simulink model "Bidirectional_AC_DC_full_control_V0_5_book"  (R2024a)
settings: Solver=VariableStepAuto  StartTime=0.0  StopTime=10.0  FixedStep=1e-6  MaxStep=1e-6  RelTol=1e-3
libraries: spsSeriesRLCBranchLib x7, simulink x7, spsBreakerLib x6, spsVoltageMeasurementLib x4, spsMosfetLib x4, spsCurrentMeasurementLib x3, slpidlib x3, spsFirstOrderFilterLib x2, spsACVoltageSourceLib x1, spsAlphaBetaZerotodq0Lib x1, spsDCVoltageSourceLib x1, sps_lib x1
settings Model: Creator=MANSY  LastModifiedBy=MANSY

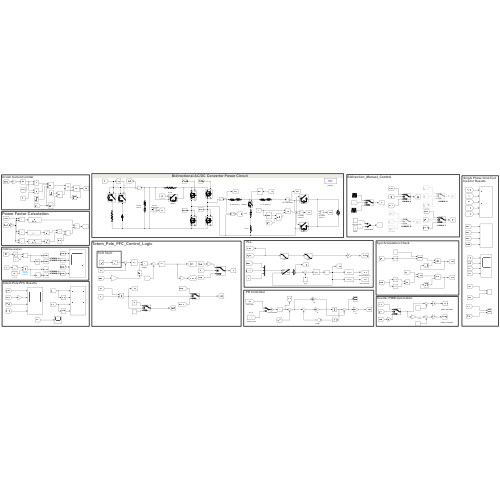
[thumbnail: Simulink's stored preview of the top-level diagram]
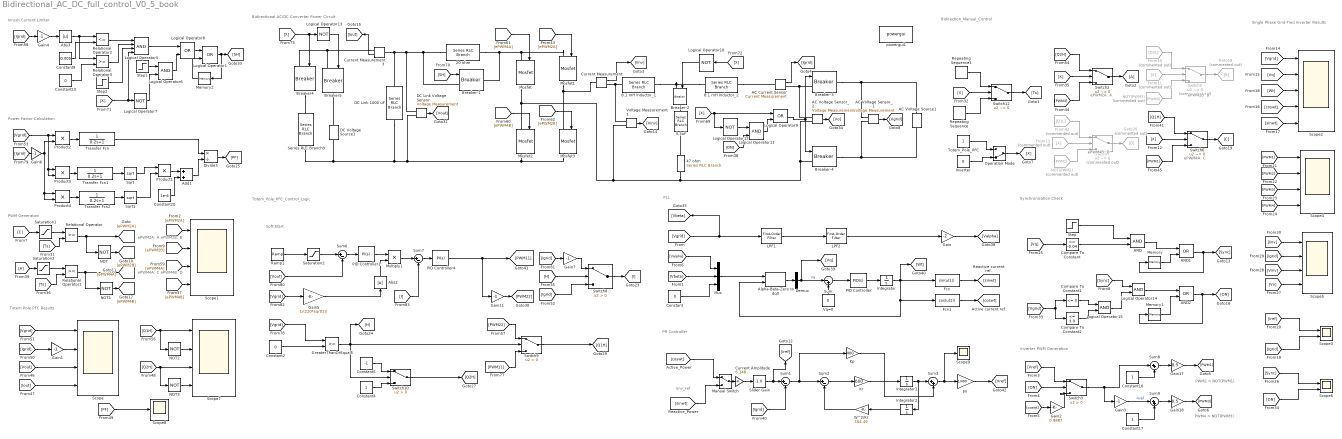
== system Bidirectional_AC_DC_full_control_V0_5_book ==
  note: Bidirectional AC/DC Converter Power Circuit
  note: Inrush Current Limiter
  note: Soft Start
  note: Power Factor Calculation
  note: Totem_Pole_PFC_Control_Logic
  note: PR Controller
  note: Synchronization Check
  note: Iinv_ref
  note: PLL
  note: Single Phase Grid-Tied
      |  Inverter Results
  note: Bidirection_Manual_Control
  note: ePWM2B: B
  note: ePWM2A: A
  note: ePWM4A: C
  note: ePWM4B: D
  note: PWM Generation
  note: PWM4 = NOT(PWM3)
  note: ePWM2A: A
      | ePWM2B: B
  note: ePWM4A: C
      | ePWM4B: D
  note: PWM2 = NOT(PWM1)
  note: Inverter PWM Generation
  note: Totem Pole PFC Results
  "          Totem_Pole_PFC" : Constant  OutDataTypeStr=boolean  SampleTime=1e-6
  20 ohm : spsSeriesRLCBranchLib/Series RLC Branch  LConnTagsString=__new0  RConnTagsString=__new0  BranchType=R  Resistance=20  Inductance=8.1e-3  SetiL0=off  InitialCurrent=0  Capacitance=1e-6  Setx0=off  InitialVoltage=0  Measurements=None
  3.3uF : spsSeriesRLCBranchLib/Series RLC Branch  LConnTagsString=__new0  RConnTagsString=__new0  BranchType=C  Resistance=30  Inductance=1e-3  SetiL0=off  InitialCurrent=0  Capacitance=3.3e-6  Setx0=off  InitialVoltage=0  Measurements=None
  47 ohm : spsSeriesRLCBranchLib/Series RLC Branch  LConnTagsString=__new0  RConnTagsString=__new0  BranchType=R  Resistance=40  Inductance=1e-3  SetiL0=off  InitialCurrent=0  Capacitance=3.3e-6  Setx0=off  InitialVoltage=0  Measurements=None
  8.1 mH Inductor_1 : spsSeriesRLCBranchLib/Series RLC Branch  LConnTagsString=__new0  RConnTagsString=__new0  BranchType=RL  Resistance=.001  Inductance=8e-3  SetiL0=off  InitialCurrent=0  Capacitance=1e-6  Setx0=off  InitialVoltage=0  Measurements=None
  8.1 mH Inductor_2 : spsSeriesRLCBranchLib/Series RLC Branch  LConnTagsString=__new0  RConnTagsString=__new0  BranchType=RL  Resistance=.001  Inductance=8e-3  SetiL0=off  InitialCurrent=0  Capacitance=1e-6  Setx0=off  InitialVoltage=0  Measurements=None
  AC Current Sensor : spsCurrentMeasurementLib/Current Measurement  PhasorSimulation=off  OutputType=Complex  PSBequivalent=0
  AC Voltage Sensor_1 : spsVoltageMeasurementLib/Voltage Measurement  PhasorSimulation=off  OutputType=Complex  PSBequivalent=0
  AC Voltage Sensor_2 : spsVoltageMeasurementLib/Voltage Measurement  PhasorSimulation=off  OutputType=Complex  PSBequivalent=0
  AC Voltage Source1 : spsACVoltageSourceLib/AC Voltage Source  Amplitude=230*sqrt(2)  Phase=0  Frequency=50  SampleTime=0  Measurements=None  BusType=swing  Pref=10e3  Qref=0  Qmin=-inf  Qmax=+inf
  AND : Logic  AllPortsSameDT=off  OutDataTypeStr=boolean
  AND1 : Logic  Operator=OR  AllPortsSameDT=off  OutDataTypeStr=boolean
  AND2 : Logic  Operator=OR  AllPortsSameDT=off  OutDataTypeStr=boolean
  Abs2 : Abs  SaturateOnIntegerOverflow=off
  Abs3 : Abs  SaturateOnIntegerOverflow=off
  Add1 : Sum
  Alpha-Beta-Zero to dq0 : spsAlphaBetaZerotodq0Lib/Alpha-Beta-Zero to dq0  Alignment=90 degrees behind phase A axis
  Breaker-{1..4} (4 alike) : spsBreakerLib/Breaker  InitialState=0  SwitchingTimes="[1/60  5/60]"  External=on  BreakerResistance=0.01  SnubberResistance=1e6  SnubberCapacitance=inf  Measurements=None  MoreParameters=on  NoBreakLoop=off
  Breaker4 : spsBreakerLib/Breaker  InitialState=0  SwitchingTimes="[1/60  5/60]"  External=on  BreakerResistance=0.01  SnubberResistance=1e6  SnubberCapacitance=inf  Measurements=None  MoreParameters=on  NoBreakLoop=off
  Breaker5 : spsBreakerLib/Breaker  InitialState=0  SwitchingTimes="[1/60  5/60]"  External=on  BreakerResistance=0.01  SnubberResistance=1e6  SnubberCapacitance=inf  Measurements=None  MoreParameters=on  NoBreakLoop=off
  Compare To Constant : simulink/Logic and Bit Operations/Compare To Constant  relop=>=  const=-0.04  OutDataTypeStr=boolean
  Compare To Constant1 : simulink/Logic and Bit Operations/Compare To Constant  relop=<=  const=0  OutDataTypeStr=boolean
  Compare To Constant2 : simulink/Logic and Bit Operations/Compare To Constant  relop=<=  const=3.0  OutDataTypeStr=boolean
  Constant : Constant  Value=0
  Constant10 : Constant  Value=0
  Constant16 : Constant
  Constant17 : Constant
  Constant2 : Constant  Value=0
  Constant20 : Constant  Value=1e-6
  Constant4 : Constant
  Constant5 : Constant  Value=-1
  Constant9 : Constant  Value=0.005
  Current Amplitude : Gain  Gain=6.148
  Current Measurement : spsCurrentMeasurementLib/Current Measurement  PhasorSimulation=off  OutputType=Complex  PSBequivalent=0
  Current Measurement3 : spsCurrentMeasurementLib/Current Measurement  PhasorSimulation=off  OutputType=Complex  PSBequivalent=0
  DC Link 1000 uF : spsSeriesRLCBranchLib/Series RLC Branch  LConnTagsString=__new0  RConnTagsString=__new0  BranchType=RC  Resistance=.0042  Inductance=1e-3  SetiL0=off  InitialCurrent=0  Capacitance=1000e-6  Setx0=off  InitialVoltage=400  Measurements=None
  DC Link Voltage Sensor : spsVoltageMeasurementLib/Voltage Measurement  PhasorSimulation=off  OutputType=Complex  PSBequivalent=0
  DC Voltage Source1 : spsDCVoltageSourceLib/DC Voltage Source  Amplitude=400  Measurements=None
  Demux : Demux  Outputs=3
  Divide3 : Product  Inputs=*/
  Fcn : Fcn  Expr=sin(u(1))
  Fcn1 : Fcn  Expr=cos(u(1))
  From10 : From  Commented=on  GotoTag=Q2L
  From11 : From  Commented=on  GotoTag=X
  From13 : From  Commented=on  GotoTag=X
  From39 : From
  From42 : From  Commented=on  GotoTag=Q1L
  Gain : Gain  Gain=-2
  Gain{1,3..4,6..7,11} (6 alike) : Gain  Gain=-1
  Gain17 : Gain  Gain=0.5
  Gain18 : Gain  Gain=0.5
  Gain2 : Gain  Gain=0.8887
  Gain5 : Gain  Gain=1/(220*sqrt(2))
  Goto18 : Goto  Commented=on  GotoTag=B
  Goto2 : Goto
  Goto20 : Goto  Commented=on  GotoTag=D
  GreaterThanOrEqual5 : RelationalOperator  OutDataTypeStr=boolean  RndMeth=Simplest  InputSameDT=off
  Integrator : Integrator
  Integrator1 : Integrator
  Integrator2 : Integrator
  Inverter : Constant  Value=0  OutDataTypeStr=boolean  SampleTime=1e-6
  Kp : Gain  Gain=400
  Kr : Gain  Gain=600
  LPF1 : spsFirstOrderFilterLib/First-Order Filter  FilterType=Lowpass  Tc=1/(2*pi*50)  Ts=0  Initialize=off  Vac_Init=[0, 0, 60]  Vdc_Init=0  PlotResponse=off  FreqRange="[0,  200,  1]"
  LPF2 : spsFirstOrderFilterLib/First-Order Filter  FilterType=Lowpass  Tc=1/(2*pi*50)  Ts=0  Initialize=off  Vac_Init=[0, 0, 60]  Vdc_Init=0  PlotResponse=off  FreqRange="[0,  200,  1]"
  Logical Operator1 : Logic  Operator=OR  AllPortsSameDT=off  OutDataTypeStr=boolean
  Logical Operator{7,10,12..13} (4 alike) : Logic  Operator=NOT  AllPortsSameDT=off  OutDataTypeStr=boolean
  Logical Operator{6,11,14..15} (4 alike) : Logic  AllPortsSameDT=off  OutDataTypeStr=boolean
  Logical Operator5 : Logic  Inputs=4  AllPortsSameDT=off  OutDataTypeStr=boolean
  Logical Operator8 : Logic  Operator=OR  AllPortsSameDT=off  OutDataTypeStr=boolean
  Logical Operator9 : Logic  Operator=OR  AllPortsSameDT=off  OutDataTypeStr=boolean
  Manual Switch : ManualSwitch
  Memory : Memory
  Memory1 : Memory
  Memory2 : Memory
  Mosfet{,1..3} (4 alike) : spsMosfetLib/Mosfet  Ron=0.1  Lon=0  Rd=0.01  Vfd=0  IC=0  Rs=1e5  Cs=inf  Measurements=on
  Multiply1 : Product
  Mux : Mux  Inputs=3
  NOT{,1..3} (4 alike) : Logic  Operator=NOT  AllPortsSameDT=off  OutDataTypeStr=boolean
  NOT(PWM1) : From  Commented=on  GotoTag=PWM2
  NOT(PWM3) : From  Commented=on  GotoTag=PWM4
  Operation Mode : ManualSwitch  CurrentSetting=0
  PID Controller : slpidlib/PID Controller  Controller=PID  Form=Parallel  TimeDomain=Continuous-time  UseExternalTs=off  SampleTime=-1  IntegratorMethod=Forward Euler  FilterMethod=Forward Euler  ControllerParametersSource=internal  P=100  I=10000  UseKiTs=off  D=0  UseExternalDerivativeSource=off  N=100  UseFilter=on  TunerSelectOption=Transfer Function Based (PID Tuner App)  InitialConditionSource=internal  InitialConditionForIntegrator=0  InitialConditionForFilter=0  DifferentiatorICPrevScaledInput=0  ExternalReset=none  TrackingMode=off  Kt=1  LimitOutput=off  SatLimitsSource=internal  UpperSaturationLimit=inf  LowerSaturationLimit=-inf  LinearizeAsGain=on  AntiWindupMode=none  Kb=1  LimitIntegrator=off  UpperIntegratorSaturationLimit=inf  LowerIntegratorSaturationLimit=-inf  POutMin=[]  POutMax=[]  IOutMin=[]  IOutMax=[]  DOutMin=[]  DOutMax=[]  NOutMin=[]  NOutMax=[]  SumOutMin=[]  SumOutMax=[]  SaturationOutMin=[]  SaturationOutMax=[]  PParamMin=[]  PParamMax=[]  IParamMin=[]  IParamMax=[]  DParamMin=[]  DParamMax=[]  NParamMin=[]  NParamMax=[]  KbParamMin=[]  KbParamMax=[]  KtParamMin=[]  KtParamMax=[]  KbOutMin=[]  KbOutMax=[]  KtOutMin=[]  KtOutMax=[]  IntegratorOutMin=[]  IntegratorOutMax=[]  FilterOutMin=[]  FilterOutMax=[]  SumI1OutMin=[]  SumI1OutMax=[]  SumI2OutMin=[]  SumI2OutMax=[]  SumI3OutMin=[]  SumI3OutMax=[]  SumI4OutMin=[]  SumI4OutMax=[]  SumDOutMin=[]  SumDOutMax=[]  DifferentiatorOutMin=[]  DifferentiatorOutMax=[]  FilterDiffOutCoefMin=[]  FilterDiffOutCoefMax=[]  ReciprocalOutMin=[]  ReciprocalOutMax=[]  SumDenOutMin=[]  SumDenOutMax=[]  SumNumOutMin=[]  SumNumOutMax=[]  DivideOutMin=[]  DivideOutMax=[]  UdiffTsProdOutMin=[]  UdiffTsProdOutMax=[]  NTsProdOutMin=[]  NTsProdOutMax=[]  UintegralTsProdOutMin=[]  UintegralTsProdOutMax=[]  UngainTsProdOutMin=[]  UngainTsProdOutMax=[]  ClampingZeroOutDataTypeStr=Inherit: Inherit via back propagation  ClampingZeroOutMin=[]  ClampingZeroOutMax=[]  FilterDenConstantOutDataTypeStr=Inherit: Inherit via back propagation  FilterDenConstantOutMin=[]  FilterDenConstantOutMax=[]  PCopyOutDataTypeStr=Inherit: Inherit via back propagation  PCopyOutMin=[]  PCopyOutMax=[]  NCopyOutDataTypeStr=Inherit: Inherit via back propagation  NCopyOutMin=[]  NCopyOutMax=[]  IntegratorContinuousStateAttributes=''  IntegratorStateMustResolveToSignalObject=off  IntegratorRTWStateStorageClass=Auto  FilterContinuousStateAttributes=''  FilterStateMustResolveToSignalObject=off  FilterRTWStateStorageClass=Auto  ParallelPVariant=InternalParameters  IdealPVariant=Disabled  IVariant=InternalParameters  DVariant=InternalParameters  IntegratorVariant=Continuous  SatVariant=Disabled  AWVariant=Passthrough  PCopyVariant=Disabled  TRVariant=Disabled  FdbkBlocksVariant=Forward  IdealPFdbkVariant=Disabled  SatFdbkVariant=Disabled  DerivativeFilterVariant=ContFilter  NVariant=InternalParameters  NCopyVariant=Disabled  FilterICVariant=InternalICsFilter  IntegratorICVariant=InternalICs  ExternalResetVariant=Disabled  TRSumVariant=Passthrough  SumFdbkVariant=Disabled  SumVariant=Sum_PID  TsampFilterVariant=InternalTs  TsampNgainVariant=Passthrough  TsampIntegralVariant=Disabled_SignalSpec  ExternalSaturationOutDataTypeStr=Inherit: Same as second input  DerivativeSourceVariant=ErrorSignal
  PID Controller1 : slpidlib/PID Controller  Controller=PI  Form=Parallel  TimeDomain=Continuous-time  UseExternalTs=off  SampleTime=-1  IntegratorMethod=Forward Euler  FilterMethod=Forward Euler  ControllerParametersSource=internal  P=.1  I=0.75  UseKiTs=off  D=0  UseExternalDerivativeSource=off  N=100  UseFilter=on  TunerSelectOption=Transfer Function Based (PID Tuner App)  InitialConditionSource=internal  InitialConditionForIntegrator=0  InitialConditionForFilter=0  DifferentiatorICPrevScaledInput=0  ExternalReset=none  TrackingMode=off  Kt=1  LimitOutput=off  SatLimitsSource=internal  UpperSaturationLimit=inf  LowerSaturationLimit=-inf  LinearizeAsGain=on  AntiWindupMode=none  Kb=1  LimitIntegrator=off  UpperIntegratorSaturationLimit=inf  LowerIntegratorSaturationLimit=-inf  POutMin=[]  POutMax=[]  IOutMin=[]  IOutMax=[]  DOutMin=[]  DOutMax=[]  NOutMin=[]  NOutMax=[]  SumOutMin=[]  SumOutMax=[]  SaturationOutMin=[]  SaturationOutMax=[]  PParamMin=[]  PParamMax=[]  IParamMin=[]  IParamMax=[]  DParamMin=[]  DParamMax=[]  NParamMin=[]  NParamMax=[]  KbParamMin=[]  KbParamMax=[]  KtParamMin=[]  KtParamMax=[]  KbOutMin=[]  KbOutMax=[]  KtOutMin=[]  KtOutMax=[]  IntegratorOutMin=[]  IntegratorOutMax=[]  FilterOutMin=[]  FilterOutMax=[]  SumI1OutMin=[]  SumI1OutMax=[]  SumI2OutMin=[]  SumI2OutMax=[]  SumI3OutMin=[]  SumI3OutMax=[]  SumI4OutMin=[]  SumI4OutMax=[]  SumDOutMin=[]  SumDOutMax=[]  DifferentiatorOutMin=[]  DifferentiatorOutMax=[]  FilterDiffOutCoefMin=[]  FilterDiffOutCoefMax=[]  ReciprocalOutMin=[]  ReciprocalOutMax=[]  SumDenOutMin=[]  SumDenOutMax=[]  SumNumOutMin=[]  SumNumOutMax=[]  DivideOutMin=[]  DivideOutMax=[]  UdiffTsProdOutMin=[]  UdiffTsProdOutMax=[]  NTsProdOutMin=[]  NTsProdOutMax=[]  UintegralTsProdOutMin=[]  UintegralTsProdOutMax=[]  UngainTsProdOutMin=[]  UngainTsProdOutMax=[]  ClampingZeroOutDataTypeStr=Inherit: Inherit via back propagation  ClampingZeroOutMin=[]  ClampingZeroOutMax=[]  FilterDenConstantOutDataTypeStr=Inherit: Inherit via back propagation  FilterDenConstantOutMin=[]  FilterDenConstantOutMax=[]  PCopyOutDataTypeStr=Inherit: Inherit via back propagation  PCopyOutMin=[]  PCopyOutMax=[]  NCopyOutDataTypeStr=Inherit: Inherit via back propagation  NCopyOutMin=[]  NCopyOutMax=[]  IntegratorContinuousStateAttributes=''  IntegratorStateMustResolveToSignalObject=off  IntegratorRTWStateStorageClass=Auto  FilterContinuousStateAttributes=''  FilterStateMustResolveToSignalObject=off  FilterRTWStateStorageClass=Auto  ParallelPVariant=InternalParameters  IdealPVariant=Disabled  IVariant=InternalParameters  DVariant=Disabled  IntegratorVariant=Continuous  SatVariant=Disabled  AWVariant=Passthrough  PCopyVariant=Disabled  TRVariant=Disabled  FdbkBlocksVariant=Forward  IdealPFdbkVariant=Disabled  SatFdbkVariant=Disabled  DerivativeFilterVariant=Disabled  NVariant=Disabled  NCopyVariant=Disabled_SignalSpec  FilterICVariant=Disabled  IntegratorICVariant=InternalICs  ExternalResetVariant=Disabled  TRSumVariant=Passthrough  SumFdbkVariant=Disabled  SumVariant=Sum_PI  TsampFilterVariant=InternalTs  TsampNgainVariant=Passthrough  TsampIntegralVariant=Disabled_SignalSpec  ExternalSaturationOutDataTypeStr=Inherit: Same as second input  DerivativeSourceVariant=Disabled
  PID Controller4 : slpidlib/PID Controller  Controller=PI  Form=Parallel  TimeDomain=Continuous-time  UseExternalTs=off  SampleTime=-1  IntegratorMethod=Forward Euler  FilterMethod=Forward Euler  ControllerParametersSource=internal  P=600  I=100  UseKiTs=off  D=0  UseExternalDerivativeSource=off  N=100  UseFilter=on  TunerSelectOption=Transfer Function Based (PID Tuner App)  InitialConditionSource=internal  InitialConditionForIntegrator=0  InitialConditionForFilter=0  DifferentiatorICPrevScaledInput=0  ExternalReset=none  TrackingMode=off  Kt=1  LimitOutput=off  SatLimitsSource=internal  UpperSaturationLimit=.99  LowerSaturationLimit=0  LinearizeAsGain=on  AntiWindupMode=none  Kb=1  LimitIntegrator=off  UpperIntegratorSaturationLimit=inf  LowerIntegratorSaturationLimit=-inf  POutMin=[]  POutMax=[]  IOutMin=[]  IOutMax=[]  DOutMin=[]  DOutMax=[]  NOutMin=[]  NOutMax=[]  SumOutMin=[]  SumOutMax=[]  SaturationOutMin=[]  SaturationOutMax=[]  PParamMin=[]  PParamMax=[]  IParamMin=[]  IParamMax=[]  DParamMin=[]  DParamMax=[]  NParamMin=[]  NParamMax=[]  KbParamMin=[]  KbParamMax=[]  KtParamMin=[]  KtParamMax=[]  KbOutMin=[]  KbOutMax=[]  KtOutMin=[]  KtOutMax=[]  IntegratorOutMin=[]  IntegratorOutMax=[]  FilterOutMin=[]  FilterOutMax=[]  SumI1OutMin=[]  SumI1OutMax=[]  SumI2OutMin=[]  SumI2OutMax=[]  SumI3OutMin=[]  SumI3OutMax=[]  SumI4OutMin=[]  SumI4OutMax=[]  SumDOutMin=[]  SumDOutMax=[]  DifferentiatorOutMin=[]  DifferentiatorOutMax=[]  FilterDiffOutCoefMin=[]  FilterDiffOutCoefMax=[]  ReciprocalOutMin=[]  ReciprocalOutMax=[]  SumDenOutMin=[]  SumDenOutMax=[]  SumNumOutMin=[]  SumNumOutMax=[]  DivideOutMin=[]  DivideOutMax=[]  UdiffTsProdOutMin=[]  UdiffTsProdOutMax=[]  NTsProdOutMin=[]  NTsProdOutMax=[]  UintegralTsProdOutMin=[]  UintegralTsProdOutMax=[]  UngainTsProdOutMin=[]  UngainTsProdOutMax=[]  ClampingZeroOutDataTypeStr=Inherit: Inherit via back propagation  ClampingZeroOutMin=[]  ClampingZeroOutMax=[]  FilterDenConstantOutDataTypeStr=Inherit: Inherit via back propagation  FilterDenConstantOutMin=[]  FilterDenConstantOutMax=[]  PCopyOutDataTypeStr=Inherit: Inherit via back propagation  PCopyOutMin=[]  PCopyOutMax=[]  NCopyOutDataTypeStr=Inherit: Inherit via back propagation  NCopyOutMin=[]  NCopyOutMax=[]  IntegratorContinuousStateAttributes=''  IntegratorStateMustResolveToSignalObject=off  IntegratorRTWStateStorageClass=Auto  FilterContinuousStateAttributes=''  FilterStateMustResolveToSignalObject=off  FilterRTWStateStorageClass=Auto  ParallelPVariant=InternalParameters  IdealPVariant=Disabled  IVariant=InternalParameters  DVariant=Disabled  IntegratorVariant=Continuous  SatVariant=Disabled  AWVariant=Passthrough  PCopyVariant=Disabled  TRVariant=Disabled  FdbkBlocksVariant=Forward  IdealPFdbkVariant=Disabled  SatFdbkVariant=Disabled  DerivativeFilterVariant=Disabled  NVariant=Disabled  NCopyVariant=Disabled_SignalSpec  FilterICVariant=Disabled  IntegratorICVariant=InternalICs  ExternalResetVariant=Disabled  TRSumVariant=Passthrough  SumFdbkVariant=Disabled  SumVariant=Sum_PI  TsampFilterVariant=InternalTs  TsampNgainVariant=Passthrough  TsampIntegralVariant=Disabled_SignalSpec  ExternalSaturationOutDataTypeStr=Inherit: Same as second input  DerivativeSourceVariant=Disabled
  Product{1..4} (4 alike) : Product
  Ramp1 : simulink/Sources/Ramp  slope=4000  start=0  InitialOutput=0
  Relational Operator : RelationalOperator  OutDataTypeStr=boolean  RndMeth=Simplest  InputSameDT=off
  Relational Operator1 : RelationalOperator  OutDataTypeStr=boolean  RndMeth=Simplest  InputSameDT=off
  Relational Operator2 : RelationalOperator  Operator=<=  OutDataTypeStr=boolean  RndMeth=Simplest  InputSameDT=off
  Relational Operator3 : RelationalOperator  OutDataTypeStr=boolean  RndMeth=Simplest  InputSameDT=off
  Repeating Sequence : simulink/Sources/Repeating Sequence  rep_seq_t=[0 1/(2*10000) 1/10000]  rep_seq_y=[0 1 0]
  Repeating Sequence1 : simulink/Sources/Repeating Sequence  rep_seq_t=[0 1/(2*100000) 1/100000]  rep_seq_y=[0 1 0]
  Saturation1 : Saturate  UpperLimit=1  LowerLimit=0
  Saturation2 : Saturate  UpperLimit=400  LowerLimit=0
  Saturation3 : Saturate  UpperLimit=1  LowerLimit=0
  Scope{,1,4..5,7} (5 alike) : Scope  NumInputPorts=4
  Scope2 : Scope  NumInputPorts=5
  Scope3 : Scope  NumInputPorts=2
  Scope6 : Scope  NumInputPorts=2
  Scope8 : Scope
  Scope9 : Scope
  Series RLC Branch9 : spsSeriesRLCBranchLib/Series RLC Branch  LConnTagsString=__new0  RConnTagsString=__new0  BranchType=R  Resistance=220  Inductance=8.1e-3  SetiL0=off  InitialCurrent=0  Capacitance=1e-6  Setx0=off  InitialVoltage=0  Measurements=None
  Slider Gain : simulink/Math Operations/Slider Gain  gain=1.0  low=0  high=1
  Sqrt : Sqrt
  Sqrt1 : Sqrt
  Step : Step  Time=0.02  SampleTime=0
  Step1 : Step  Time=0.005  SampleTime=0
  Step2 : Step  Time=0.13  SampleTime=0
  Sum : Sum  Inputs=|-+
  Sum{1..2,6..7} (4 alike) : Sum  Inputs=|+-
  Sum3 : Sum  Inputs=|++
  Sum8 : Sum  Inputs=|++
  Sum9 : Sum  Inputs=|++
  Switch{3,8..10} (4 alike) : Switch  Criteria=u2 > Threshold  SaturateOnIntegerOverflow=off  InputSameDT=off
  Switch12 : Switch  Criteria=u2 ~= 0  SaturateOnIntegerOverflow=off  InputSameDT=off
  Switch2 : Switch  Criteria=u2 ~= 0  SaturateOnIntegerOverflow=off  InputSameDT=off
  Switch5 : Switch  Commented=on  Criteria=u2 ~= 0  SaturateOnIntegerOverflow=off  InputSameDT=off
  Switch6 : Switch  Criteria=u2 ~= 0  SaturateOnIntegerOverflow=off  InputSameDT=off
  Switch7 : Switch  Commented=on  Criteria=u2 ~= 0  SaturateOnIntegerOverflow=off  InputSameDT=off
  Transfer Fcn : TransferFcn  Denominator=[0.2 1]
  Transfer Fcn1 : TransferFcn  Denominator=[0.2 1]
  Transfer Fcn2 : TransferFcn  Denominator=[0.2 1]
  Voltage Measurement1 : spsVoltageMeasurementLib/Voltage Measurement  PhasorSimulation=off  OutputType=Complex  PSBequivalent=0
  Vq=0 : Constant  Value=0
  W^2/Kr : Gain  Gain=164.49
  powergui1 : sps_lib/powergui  Priority=1  SimulationMode=Discrete  SampleTime=1e-6  frequency=60  Iterations=50  frequencyindice=0  Pbase=100e6  ErrMax=1e-4  UnitsV=kV  UnitsW=MW  buscounter=0  FunctionMessages=off  echomessages=off  EnableUseOfTLC=off  CurrentSourceSwitches=off  DisableSnubberDevices=off  DisableRonSwitches=off  DisableVfSwitches=off  DisplayEquations=off  AutomaticDiscreteSolvers=off  SolverType=Tustin/Backward Euler (TBE)  Interpol=off  ExternalGateDelay=off  methode=off  Ts=100  x0status=blocks  SPID=on  SwTol=0  HookPort=off  NonlinearTolerance=1e-4  nMaxIteration=100  ContinueOnMaxIteration=off  RestoreLinks=warning  ResistiveCurrentMeasurement=off  Frange=[0:2:500]  Ylog=off  Xlog=on  ShowGrid=off  save=off  variable=ZData  structure=0  ZoomFFT=off  StartTime=0.0  cycles=1  DisplayStyle=1  fundamental=60  FreqAxis=off  MaxFrequency=1000  frequencyindicesteady=1  RmsSteady=1  display=off
  pu : Gain  Gain=1/400
  wires:
  [ePWM2B] -> Mosfet3/1
  Voltage Measurement1/1 -> [Vinv]
  [ePWM2A] -> Mosfet1/1
  Step1/1 -> Logical Operator6/1
  AC Voltage Sensor_1/1 -> [Vgrid]
  Relational Operator2/1 -> Logical Operator5/1
  Logical Operator12/1 -> Logical Operator11/1
  Constant9/1 -> Relational Operator2/2
  Gain4/1 -> Abs3/1
  [X] -> Logical Operator5/4, Logical Operator7/1
  [SH] -> Breaker-1/1
  Abs3/1 -> Relational Operator3/1, Relational Operator2/1
  [Igrid] -> Gain4/1
  [ePWM4A] -> Mosfet/1
  Constant10/1 -> Relational Operator3/2
  Logical Operator13/1 -> Breaker5/1
  Logical Operator5/1 -> Logical Operator8/1
  AC Voltage Sensor_2/1 -> [Vo]
  Relational Operator3/1 -> Logical Operator5/2
  Step2/1 -> Logical Operator5/3
  [X] -> Breaker4/1, Logical Operator13/1
  Logical Operator11/1 -> Logical Operator9/2
  Logical Operator6/1 -> Logical Operator8/2
  [X] -> Logical Operator9/1, Logical Operator12/1
  [ON] -> Logical Operator11/2
  [ePWM4B] -> Mosfet2/1
  [X] -> Logical Operator10/1
  Logical Operator10/1 -> Breaker-2/1
  Current Measurement/1 -> [Iinv]
  Logical Operator9/1 -> Breaker-4/1, Breaker-3/1
  AC Current Sensor/1 -> [Igrid]
  Current Measurement3/1 -> [Iout]
  DC Link Voltage Sensor/1 -> [Vout]
  Logical Operator7/1 -> Logical Operator6/2
  Switch9/1 -> [Q1H]
  Transfer Fcn/1 -> Divide3/1
  Constant4/1 -> Switch10/3
  [Igrid] -> Switch8/3
  Gain11/1 -> [PWM22]
  Transfer Fcn2/1 -> Sqrt1/1
  Gain7/1 -> Switch8/1
  Product1/1 -> Add1/1
  Abs2/1 -> Multiply1/2
  Gain5/1 -> Abs2/1
  Ramp1/1 -> Saturation2/1
  [PWM22] -> Switch9/1
  Product4/1 -> Transfer Fcn2/1
  Constant20/1 -> Add1/2
  Divide3/1 -> [PF]
  Sqrt/1 -> Product1/1
  Switch10/1 -> [Q2H]
  [Igrid] -> Gain7/1
  [Vgrid] -> Product2/1, Product3/2, Product3/1
  Transfer Fcn1/1 -> Sqrt/1
  [H] -> Switch8/2
  [I] -> Sum7/2
  Product2/1 -> Transfer Fcn/1
  PID Controller4/1 -> Gain11/1, [PWM11]
  Switch8/1 -> [I]
  Product3/1 -> Transfer Fcn1/1
  Saturation2/1 -> Sum6/1
  GreaterThanOrEqual5/1 -> Switch10/2, Switch9/2, [H]
  Constant2/1 -> GreaterThanOrEqual5/2
  Multiply1/1 -> Sum7/1
  [PWM11] -> Switch9/3
  Constant5/1 -> Switch10/1
  [Vout] -> Sum6/2
  Sum7/1 -> PID Controller4/1
  [Igrid] -> Gain6/1
  [Vgrid] -> Gain5/1
  Sqrt1/1 -> Product1/2
  PID Controller1/1 -> Multiply1/1
  Sum6/1 -> PID Controller1/1
  Add1/1 -> Divide3/2
  [Vgrid] -> GreaterThanOrEqual5/1
  [Vgrid] -> Scope2/1
  Logical Operator15/1 -> Logical Operator14/2
  PID Controller/1 -> Integrator/1
  [Valpha] -> Mux/1
  [Igrid] -> Scope3/2
  Integrator1/1 -> Integrator2/1, Sum3/1
  [Vq] -> Scope2/2
  Memory1/1 -> AND2/2
  Constant/1 -> Mux/3
  AND1/1 -> [Sync], Memory/1
  [Iref] -> Scope3/1
  Compare To Constant/1 -> AND/2
  [Sync] -> Logical Operator14/1
  [Vinv] -> Scope5/3
  Fcn/1 -> [sinwt]
  Mux/1 -> Alpha-Beta-Zero to dq0/1
  Memory/1 -> AND1/2
  pu/1 -> [Vref]
  [sinwt] -> Scope2/5
  AND/1 -> AND1/1
  Gain/1 -> [Valpha]
  Current Amplitude/1 -> Slider Gain/1
  Integrator/1 -> [Wt], Fcn/1, Fcn1/1, Alpha-Beta-Zero to dq0/2
  Manual Switch/1 -> Current Amplitude/1
  [PWM2] -> Scope4/2
  [PWM1] -> Scope4/1
  [PWM3] -> Scope4/3
  Alpha-Beta-Zero to dq0/1 -> Demux/1
  Sum2/1 -> Kr/1
  [Wt] -> Scope2/3
  [Sync] -> Scope6/1
  Sum/1 -> PID Controller/1
  Step/1 -> AND/1
  [coswt] -> Manual Switch/1
  LPF2/1 -> Gain/1
  Sum1/1 -> Sum2/1, Kp/1
  [ON] -> Scope6/2
  Kr/1 -> Integrator1/1
  [Vgrid] -> Compare To Constant1/1, Compare To Constant2/1
  [Vbeta] -> Mux/2
  [Iinv] -> Scope5/1
  Integrator2/1 -> W^2/Kr/1
  [sinwt] -> Manual Switch/2
  [Vgrid] -> [Vbeta], LPF1/1
  [PWM4] -> Scope4/4
  Kp/1 -> Sum3/2
  W^2/Kr/1 -> Sum2/2
  [coswt] -> Scope2/4
  Slider Gain/1 -> [Iref], Sum1/1
  AND2/1 -> Memory1/1, [ON]
  Logical Operator14/1 -> AND2/1
  LPF1/1 -> LPF2/1
  [Vo] -> Scope5/4
  Compare To Constant1/1 -> Logical Operator15/1
  Sum3/1 -> Scope9/1, pu/1
  [Igrid] -> Scope5/2
  Vq=0/1 -> Sum/2
  [Igrid] -> Sum1/2
  Fcn1/1 -> [coswt]
  [Vq] -> Compare To Constant/1
  Compare To Constant2/1 -> Logical Operator15/2
  Demux/2 -> Sum/1, [Vq]  "Vq"
  [PWM3] -> Switch2/3
  Operation Mode/1 -> [X]
  Switch6/1 -> [C]
  Switch2/1 -> Goto2/1
  [Q2H] -> Switch2/1
  NOT(PWM3)/1 -> Switch5/3
  From10/1 -> Switch5/1
  From42/1 -> Switch7/1
  Switch12/1 -> [Ts]
  [X] -> Switch6/2
  Repeating Sequence/1 -> Switch12/3
  Switch5/1 -> Goto18/1
  [PWM1] -> Switch6/3
  NOT(PWM1)/1 -> Switch7/3
  From13/1 -> Switch7/2
  Inverter/1 -> Operation Mode/2
  From11/1 -> Switch5/2
  [Q1H] -> Switch6/1
  [X] -> Switch12/2
  [X] -> Switch2/2
  Switch7/1 -> Goto20/1
  "          Totem_Pole_PFC"/1 -> Operation Mode/1
  Repeating Sequence1/1 -> Switch12/1
  Gain18/1 -> [PWM3]
  Gain17/1 -> [PWM1]
  Constant16/1 -> Sum8/2
  Sum8/1 -> Gain17/1
  [ON] -> Switch3/2
  [coswt] -> Gain2/1
  [Vref] -> Switch3/1
  Gain2/1 -> Switch3/3
  Switch3/1 -> Sum8/1, Gain3/1
  Sum9/1 -> Gain18/1
  Constant17/1 -> Sum9/2
  [C] -> Saturation1/1
  Gain3/1 -> Sum9/1  "-Vref"
  Saturation1/1 -> Relational Operator/1
  [Ts] -> Relational Operator/2
  [Ts] -> Relational Operator1/2
  Saturation3/1 -> Relational Operator1/1
  From39/1 -> Saturation3/1
  Relational Operator/1 -> NOT/1, [ePWM2A]
  NOT/1 -> [ePWM2B]
  NOT1/1 -> [ePWM4B]
  [ePWM2A] -> Scope1/1
  [ePWM2B] -> Scope1/2
  [ePWM4A] -> Scope1/3
  [ePWM4B] -> Scope1/4
  [PF] -> Scope8/1
  [Q2H] -> NOT3/1, Scope7/3
  [Iout] -> Scope/4
  NOT2/1 -> Scope7/2
  [Vout] -> Scope/3
  NOT3/1 -> Scope7/4
  Gain1/1 -> Scope/2
  [Q1H] -> NOT2/1, Scope7/1
  [Igrid] -> Gain1/1
  [Vgrid] -> Scope/1
  Gain6/1 -> Product2/2, Product4/2, Product4/1
  Logical Operator8/1 -> Logical Operator1/1
  Logical Operator1/1 -> Memory2/1, [SH]
  Memory2/1 -> Logical Operator1/2
  Relational Operator1/1 -> NOT1/1, [ePWM4A]
  connections:
  20 ohm/LConn1 -- DC Link 1000 uF/LConn1 -- Current Measurement3/LConn1 -- DC Link Voltage Sensor/LConn1 -- Breaker-1/LConn1
  AC Voltage Sensor_1/LConn1 -- AC Voltage Source1/RConn1 -- Breaker-3/RConn1
  Current Measurement3/RConn1 -- Breaker5/LConn1 -- Breaker4/LConn1
  8.1 mH Inductor_2/LConn1 -- 8.1 mH Inductor_1/RConn1 -- Breaker-2/LConn1
  AC Voltage Sensor_2/LConn2 -- Breaker-4/LConn1 -- Voltage Measurement1/LConn2 -- Mosfet/RConn1 -- Mosfet2/LConn1 -- 47 ohm/RConn1
  DC Voltage Source1/LConn1 -- DC Link 1000 uF/RConn1 -- DC Link Voltage Sensor/LConn2 -- Mosfet3/RConn1 -- Mosfet2/RConn1 -- Series RLC Branch9/RConn1
  AC Voltage Source1/LConn1 -- AC Voltage Sensor_1/LConn2 -- Breaker-4/RConn1
  AC Current Sensor/RConn1 -- Breaker-3/LConn1 -- AC Voltage Sensor_2/LConn1
  Mosfet1/LConn1 -- 20 ohm/RConn1 -- Breaker-1/RConn1 -- Mosfet/LConn1
  Voltage Measurement1/LConn1 -- 8.1 mH Inductor_1/LConn1 -- Current Measurement/RConn1
  8.1 mH Inductor_2/RConn1 -- AC Current Sensor/LConn1
  Breaker-2/RConn1 -- 3.3uF/LConn1
  Breaker4/RConn1 -- Series RLC Branch9/LConn1
  Mosfet1/RConn1 -- Current Measurement/LConn1 -- Mosfet3/LConn1
  DC Voltage Source1/RConn1 -- Breaker5/RConn1
  47 ohm/LConn1 -- 3.3uF/RConn1
